simulink model "solar_pv_protected_c07_circuit"  (R2026b)
settings: Solver=VariableStepAuto
model workspace (MAT data in the model file):
  candidate_owner = 'pv_protection_integration_20261023_r01'
  solar_edit_metadata : object (value not decoded)
libraries: fl_lib x149, ee_lib x16, ltc4364demo_lib x3, batteryecm_lib x1, solarprotect_lib x1
(part 13 of 16)

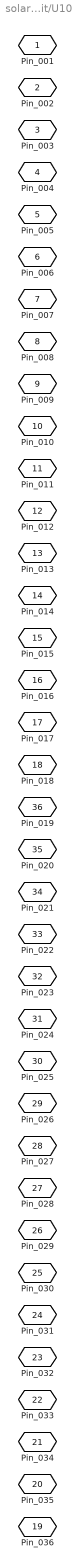
== system solar_pv_protected_c07_circuit/U10 ==
  Pin_001 : PMIOPort  Description=|  Side=Left  ConnectionType=Connection: foundation.electrical.electrical
      | 識別名　　　　　　　; Pin_001
      | 種別　　　　　　　　; Simscape Connection Port（階層境界の物理端子）
      | 所属部品　　　　　　; U10
      | 配置目的　　　　　　; 内部の電気ノードを、この外箱の外側の対応端子へ引き出す。
      | 対応端子　　　　　　; lconn:1／1番 GNDP
      | 接続ラベル　　　　　; GND、PROT_RETURN
      | モデルの範囲　　　　; 実部品を1個追加する表現ではない。端子自体に増幅・遮断・測定機能を持たない。
      | 端子番号の注意　　　; Connection Portの番号は外箱内の対応番号であり、実パッケージのピン番号とは区別する。
      | 確認の範囲　　　　　; 実ポートと階層対応による静的接続の説明。電気特性の再現性は所属部品の説明を参照する。
      | 
      | 従来の補足　　　　　; 以前のDescriptionを以下に保持する。
      | Physical U10 pin 1 / GNDP
      | 
      | 【この説明欄の略語・記号】
      | 用語1　　　　　　　 ; IC：Integrated Circuit（集積回路）。複数の電子素子と機能を小さな半導体チップに集積した部品。
      | 用語2　　　　　　　 ; MOSFET：Metal-Oxide-Semiconductor Field-Effect Transistor（金属・酸化膜・半導体構造の電界効果トランジスタ）。ゲートとソースの電圧でドレインとソースの導通を制御する素子。N-MOSはNチャネル型を表す。
      | 用語3　　　　　　　 ; GND：Ground（回路の基準電位・電流帰路）。この図の共通基準。保護接地や大地への接続を意味するとは限らない。
      | 用語4　　　　　　　 ; VCC/VDD/VEE/VS：ICの電源端子名。文字の歴史的な由来を現在の接続機能へ当てはめない。現回路のVEEはU8/U10では浮動基準SW、U9ではGND。各電圧・基準は端子と接続を参照する。
      | 用語5　　　　　　　 ; GNDP：U10の一次側電源の基準端子。絶縁電源の入力側GND。二次側基準VEE=SWと直接同一の導体ではない。
      | 用語6　　　　　　　 ; SW：Switching Node（スイッチング点）。主電力段の上下MOSFETとL1がつながる、電圧が高速に切り替わる点。GNDとは別電位。
      | 用語7　　　　　　　 ; PROT_RETURN：保護回路の共通帰路。PROTはProtection（保護）、RETURNは帰路。プロトタイプの略ではなく、現回路では共通GNDへつながる。
  Pin_002 : PMIOPort  Description=|  Port=2  Side=Left  ConnectionType=Connection: foundation.electrical.electrical
      | 識別名　　　　　　　; Pin_002
      | 種別　　　　　　　　; Simscape Connection Port（階層境界の物理端子）
      | 所属部品　　　　　　; U10
      | 配置目的　　　　　　; 内部の電気ノードを、この外箱の外側の対応端子へ引き出す。
      | 対応端子　　　　　　; lconn:2／2番 GNDP
      | 接続ラベル　　　　　; GND、PROT_RETURN
      | モデルの範囲　　　　; 実部品を1個追加する表現ではない。端子自体に増幅・遮断・測定機能を持たない。
      | 端子番号の注意　　　; Connection Portの番号は外箱内の対応番号であり、実パッケージのピン番号とは区別する。
      | 確認の範囲　　　　　; 実ポートと階層対応による静的接続の説明。電気特性の再現性は所属部品の説明を参照する。
      | 
      | 従来の補足　　　　　; 以前のDescriptionを以下に保持する。
      | Physical U10 pin 2 / GNDP
      | 
      | 【この説明欄の略語・記号】
      | 用語1　　　　　　　 ; IC：Integrated Circuit（集積回路）。複数の電子素子と機能を小さな半導体チップに集積した部品。
      | 用語2　　　　　　　 ; MOSFET：Metal-Oxide-Semiconductor Field-Effect Transistor（金属・酸化膜・半導体構造の電界効果トランジスタ）。ゲートとソースの電圧でドレインとソースの導通を制御する素子。N-MOSはNチャネル型を表す。
      | 用語3　　　　　　　 ; GND：Ground（回路の基準電位・電流帰路）。この図の共通基準。保護接地や大地への接続を意味するとは限らない。
      | 用語4　　　　　　　 ; VCC/VDD/VEE/VS：ICの電源端子名。文字の歴史的な由来を現在の接続機能へ当てはめない。現回路のVEEはU8/U10では浮動基準SW、U9ではGND。各電圧・基準は端子と接続を参照する。
      | 用語5　　　　　　　 ; GNDP：U10の一次側電源の基準端子。絶縁電源の入力側GND。二次側基準VEE=SWと直接同一の導体ではない。
      | 用語6　　　　　　　 ; SW：Switching Node（スイッチング点）。主電力段の上下MOSFETとL1がつながる、電圧が高速に切り替わる点。GNDとは別電位。
      | 用語7　　　　　　　 ; PROT_RETURN：保護回路の共通帰路。PROTはProtection（保護）、RETURNは帰路。プロトタイプの略ではなく、現回路では共通GNDへつながる。
  Pin_003 : PMIOPort  Description=|  Port=3  Side=Left  ConnectionType=Connection: foundation.electrical.electrical
      | 識別名　　　　　　　; Pin_003
      | 種別　　　　　　　　; Simscape Connection Port（階層境界の物理端子）
      | 所属部品　　　　　　; U10
      | 配置目的　　　　　　; 内部の電気ノードを、この外箱の外側の対応端子へ引き出す。
      | 対応端子　　　　　　; lconn:3／3番 PG
      | 接続ラベル　　　　　; BIAS_PG
      | モデルの範囲　　　　; 実部品を1個追加する表現ではない。端子自体に増幅・遮断・測定機能を持たない。
      | 端子番号の注意　　　; Connection Portの番号は外箱内の対応番号であり、実パッケージのピン番号とは区別する。
      | 確認の範囲　　　　　; 実ポートと階層対応による静的接続の説明。電気特性の再現性は所属部品の説明を参照する。
      | 
      | 従来の補足　　　　　; 以前のDescriptionを以下に保持する。
      | Physical U10 pin 3 / PG
      | 
      | 【この説明欄の略語・記号】
      | 用語1　　　　　　　 ; IC：Integrated Circuit（集積回路）。複数の電子素子と機能を小さな半導体チップに集積した部品。
      | 用語2　　　　　　　 ; PG：Power Good（電源状態通知）。電源出力が規定状態にあるかを知らせる信号。プルアップ条件と実際の通知条件は対象ICの説明で確認する。
  Pin_004 : PMIOPort  Description=|  Port=4  Side=Left  ConnectionType=Connection: foundation.electrical.electrical
      | 識別名　　　　　　　; Pin_004
      | 種別　　　　　　　　; Simscape Connection Port（階層境界の物理端子）
      | 所属部品　　　　　　; U10
      | 配置目的　　　　　　; 内部の電気ノードを、この外箱の外側の対応端子へ引き出す。
      | 対応端子　　　　　　; lconn:4／4番 ENA
      | 接続ラベル　　　　　; BIAS_EN
      | モデルの範囲　　　　; 実部品を1個追加する表現ではない。端子自体に増幅・遮断・測定機能を持たない。
      | 端子番号の注意　　　; Connection Portの番号は外箱内の対応番号であり、実パッケージのピン番号とは区別する。
      | 確認の範囲　　　　　; 実ポートと階層対応による静的接続の説明。電気特性の再現性は所属部品の説明を参照する。
      | 
      | 従来の補足　　　　　; 以前のDescriptionを以下に保持する。
      | Physical U10 pin 4 / ENA
      | 
      | 【この説明欄の略語・記号】
      | 用語1　　　　　　　 ; EN：Enable（動作許可）。対象機能の動作を許可する信号。端子ごとの有効レベルや接続状態に従う。
  Pin_005 : PMIOPort  Description=|  Port=5  Side=Left  ConnectionType=Connection: foundation.electrical.electrical
      | 識別名　　　　　　　; Pin_005
      | 種別　　　　　　　　; Simscape Connection Port（階層境界の物理端子）
      | 所属部品　　　　　　; U10
      | 配置目的　　　　　　; 内部の電気ノードを、この外箱の外側の対応端子へ引き出す。
      | 対応端子　　　　　　; lconn:5／5番 GNDP
      | 接続ラベル　　　　　; GND、PROT_RETURN
      | モデルの範囲　　　　; 実部品を1個追加する表現ではない。端子自体に増幅・遮断・測定機能を持たない。
      | 端子番号の注意　　　; Connection Portの番号は外箱内の対応番号であり、実パッケージのピン番号とは区別する。
      | 確認の範囲　　　　　; 実ポートと階層対応による静的接続の説明。電気特性の再現性は所属部品の説明を参照する。
      | 
      | 従来の補足　　　　　; 以前のDescriptionを以下に保持する。
      | Physical U10 pin 5 / GNDP
      | 
      | 【この説明欄の略語・記号】
      | 用語1　　　　　　　 ; IC：Integrated Circuit（集積回路）。複数の電子素子と機能を小さな半導体チップに集積した部品。
      | 用語2　　　　　　　 ; MOSFET：Metal-Oxide-Semiconductor Field-Effect Transistor（金属・酸化膜・半導体構造の電界効果トランジスタ）。ゲートとソースの電圧でドレインとソースの導通を制御する素子。N-MOSはNチャネル型を表す。
      | 用語3　　　　　　　 ; GND：Ground（回路の基準電位・電流帰路）。この図の共通基準。保護接地や大地への接続を意味するとは限らない。
      | 用語4　　　　　　　 ; VCC/VDD/VEE/VS：ICの電源端子名。文字の歴史的な由来を現在の接続機能へ当てはめない。現回路のVEEはU8/U10では浮動基準SW、U9ではGND。各電圧・基準は端子と接続を参照する。
      | 用語5　　　　　　　 ; GNDP：U10の一次側電源の基準端子。絶縁電源の入力側GND。二次側基準VEE=SWと直接同一の導体ではない。
      | 用語6　　　　　　　 ; SW：Switching Node（スイッチング点）。主電力段の上下MOSFETとL1がつながる、電圧が高速に切り替わる点。GNDとは別電位。
      | 用語7　　　　　　　 ; PROT_RETURN：保護回路の共通帰路。PROTはProtection（保護）、RETURNは帰路。プロトタイプの略ではなく、現回路では共通GNDへつながる。
  Pin_006 : PMIOPort  Description=|  Port=6  Side=Left  ConnectionType=Connection: foundation.electrical.electrical
      | 識別名　　　　　　　; Pin_006
      | 種別　　　　　　　　; Simscape Connection Port（階層境界の物理端子）
      | 所属部品　　　　　　; U10
      | 配置目的　　　　　　; 内部の電気ノードを、この外箱の外側の対応端子へ引き出す。
      | 対応端子　　　　　　; lconn:6／6番 VIN
      | 接続ラベル　　　　　; P12
      | モデルの範囲　　　　; 実部品を1個追加する表現ではない。端子自体に増幅・遮断・測定機能を持たない。
      | 端子番号の注意　　　; Connection Portの番号は外箱内の対応番号であり、実パッケージのピン番号とは区別する。
      | 確認の範囲　　　　　; 実ポートと階層対応による静的接続の説明。電気特性の再現性は所属部品の説明を参照する。
      | 
      | 従来の補足　　　　　; 以前のDescriptionを以下に保持する。
      | Physical U10 pin 6 / VIN
      | 
      | 【この説明欄の略語・記号】
      | 用語1　　　　　　　 ; VIN/VOUT：入力電圧・出力電圧を表す端子／ネット名。INは入力、OUTは出力。電源変換器の電力端子なのか、検出用端子なのかは対象部品によって異なるため、端子と接続の説明に従う。
  Pin_007 : PMIOPort  Description=|  Port=7  Side=Left  ConnectionType=Connection: foundation.electrical.electrical
      | 識別名　　　　　　　; Pin_007
      | 種別　　　　　　　　; Simscape Connection Port（階層境界の物理端子）
      | 所属部品　　　　　　; U10
      | 配置目的　　　　　　; 内部の電気ノードを、この外箱の外側の対応端子へ引き出す。
      | 対応端子　　　　　　; lconn:7／7番 VIN
      | 接続ラベル　　　　　; P12
      | モデルの範囲　　　　; 実部品を1個追加する表現ではない。端子自体に増幅・遮断・測定機能を持たない。
      | 端子番号の注意　　　; Connection Portの番号は外箱内の対応番号であり、実パッケージのピン番号とは区別する。
      | 確認の範囲　　　　　; 実ポートと階層対応による静的接続の説明。電気特性の再現性は所属部品の説明を参照する。
      | 
      | 従来の補足　　　　　; 以前のDescriptionを以下に保持する。
      | Physical U10 pin 7 / VIN
      | 
      | 【この説明欄の略語・記号】
      | 用語1　　　　　　　 ; VIN/VOUT：入力電圧・出力電圧を表す端子／ネット名。INは入力、OUTは出力。電源変換器の電力端子なのか、検出用端子なのかは対象部品によって異なるため、端子と接続の説明に従う。
  Pin_008 : PMIOPort  Description=|  Port=8  Side=Left  ConnectionType=Connection: foundation.electrical.electrical
      | 識別名　　　　　　　; Pin_008
      | 種別　　　　　　　　; Simscape Connection Port（階層境界の物理端子）
      | 所属部品　　　　　　; U10
      | 配置目的　　　　　　; 内部の電気ノードを、この外箱の外側の対応端子へ引き出す。
      | 対応端子　　　　　　; lconn:8／8番 GNDP
      | 接続ラベル　　　　　; GND、PROT_RETURN
      | モデルの範囲　　　　; 実部品を1個追加する表現ではない。端子自体に増幅・遮断・測定機能を持たない。
      | 端子番号の注意　　　; Connection Portの番号は外箱内の対応番号であり、実パッケージのピン番号とは区別する。
      | 確認の範囲　　　　　; 実ポートと階層対応による静的接続の説明。電気特性の再現性は所属部品の説明を参照する。
      | 
      | 従来の補足　　　　　; 以前のDescriptionを以下に保持する。
      | Physical U10 pin 8 / GNDP
      | 
      | 【この説明欄の略語・記号】
      | 用語1　　　　　　　 ; IC：Integrated Circuit（集積回路）。複数の電子素子と機能を小さな半導体チップに集積した部品。
      | 用語2　　　　　　　 ; MOSFET：Metal-Oxide-Semiconductor Field-Effect Transistor（金属・酸化膜・半導体構造の電界効果トランジスタ）。ゲートとソースの電圧でドレインとソースの導通を制御する素子。N-MOSはNチャネル型を表す。
      | 用語3　　　　　　　 ; GND：Ground（回路の基準電位・電流帰路）。この図の共通基準。保護接地や大地への接続を意味するとは限らない。
      | 用語4　　　　　　　 ; VCC/VDD/VEE/VS：ICの電源端子名。文字の歴史的な由来を現在の接続機能へ当てはめない。現回路のVEEはU8/U10では浮動基準SW、U9ではGND。各電圧・基準は端子と接続を参照する。
      | 用語5　　　　　　　 ; GNDP：U10の一次側電源の基準端子。絶縁電源の入力側GND。二次側基準VEE=SWと直接同一の導体ではない。
      | 用語6　　　　　　　 ; SW：Switching Node（スイッチング点）。主電力段の上下MOSFETとL1がつながる、電圧が高速に切り替わる点。GNDとは別電位。
      | 用語7　　　　　　　 ; PROT_RETURN：保護回路の共通帰路。PROTはProtection（保護）、RETURNは帰路。プロトタイプの略ではなく、現回路では共通GNDへつながる。
  Pin_009 : PMIOPort  Description=|  Port=9  Side=Left  ConnectionType=Connection: foundation.electrical.electrical
      | 識別名　　　　　　　; Pin_009
      | 種別　　　　　　　　; Simscape Connection Port（階層境界の物理端子）
      | 所属部品　　　　　　; U10
      | 配置目的　　　　　　; 内部の電気ノードを、この外箱の外側の対応端子へ引き出す。
      | 対応端子　　　　　　; lconn:9／9番 GNDP
      | 接続ラベル　　　　　; GND、PROT_RETURN
      | モデルの範囲　　　　; 実部品を1個追加する表現ではない。端子自体に増幅・遮断・測定機能を持たない。
      | 端子番号の注意　　　; Connection Portの番号は外箱内の対応番号であり、実パッケージのピン番号とは区別する。
      | 確認の範囲　　　　　; 実ポートと階層対応による静的接続の説明。電気特性の再現性は所属部品の説明を参照する。
      | 
      | 従来の補足　　　　　; 以前のDescriptionを以下に保持する。
      | Physical U10 pin 9 / GNDP
      | 
      | 【この説明欄の略語・記号】
      | 用語1　　　　　　　 ; IC：Integrated Circuit（集積回路）。複数の電子素子と機能を小さな半導体チップに集積した部品。
      | 用語2　　　　　　　 ; MOSFET：Metal-Oxide-Semiconductor Field-Effect Transistor（金属・酸化膜・半導体構造の電界効果トランジスタ）。ゲートとソースの電圧でドレインとソースの導通を制御する素子。N-MOSはNチャネル型を表す。
      | 用語3　　　　　　　 ; GND：Ground（回路の基準電位・電流帰路）。この図の共通基準。保護接地や大地への接続を意味するとは限らない。
      | 用語4　　　　　　　 ; VCC/VDD/VEE/VS：ICの電源端子名。文字の歴史的な由来を現在の接続機能へ当てはめない。現回路のVEEはU8/U10では浮動基準SW、U9ではGND。各電圧・基準は端子と接続を参照する。
      | 用語5　　　　　　　 ; GNDP：U10の一次側電源の基準端子。絶縁電源の入力側GND。二次側基準VEE=SWと直接同一の導体ではない。
      | 用語6　　　　　　　 ; SW：Switching Node（スイッチング点）。主電力段の上下MOSFETとL1がつながる、電圧が高速に切り替わる点。GNDとは別電位。
      | 用語7　　　　　　　 ; PROT_RETURN：保護回路の共通帰路。PROTはProtection（保護）、RETURNは帰路。プロトタイプの略ではなく、現回路では共通GNDへつながる。
  Pin_010 : PMIOPort  Description=|  Port=10  Side=Left  ConnectionType=Connection: foundation.electrical.electrical
      | 識別名　　　　　　　; Pin_010
      | 種別　　　　　　　　; Simscape Connection Port（階層境界の物理端子）
      | 所属部品　　　　　　; U10
      | 配置目的　　　　　　; 内部の電気ノードを、この外箱の外側の対応端子へ引き出す。
      | 対応端子　　　　　　; lconn:10／10番 GNDP
      | 接続ラベル　　　　　; GND、PROT_RETURN
      | モデルの範囲　　　　; 実部品を1個追加する表現ではない。端子自体に増幅・遮断・測定機能を持たない。
      | 端子番号の注意　　　; Connection Portの番号は外箱内の対応番号であり、実パッケージのピン番号とは区別する。
      | 確認の範囲　　　　　; 実ポートと階層対応による静的接続の説明。電気特性の再現性は所属部品の説明を参照する。
      | 
      | 従来の補足　　　　　; 以前のDescriptionを以下に保持する。
      | Physical U10 pin 10 / GNDP
      | 
      | 【この説明欄の略語・記号】
      | 用語1　　　　　　　 ; IC：Integrated Circuit（集積回路）。複数の電子素子と機能を小さな半導体チップに集積した部品。
      | 用語2　　　　　　　 ; MOSFET：Metal-Oxide-Semiconductor Field-Effect Transistor（金属・酸化膜・半導体構造の電界効果トランジスタ）。ゲートとソースの電圧でドレインとソースの導通を制御する素子。N-MOSはNチャネル型を表す。
      | 用語3　　　　　　　 ; GND：Ground（回路の基準電位・電流帰路）。この図の共通基準。保護接地や大地への接続を意味するとは限らない。
      | 用語4　　　　　　　 ; VCC/VDD/VEE/VS：ICの電源端子名。文字の歴史的な由来を現在の接続機能へ当てはめない。現回路のVEEはU8/U10では浮動基準SW、U9ではGND。各電圧・基準は端子と接続を参照する。
      | 用語5　　　　　　　 ; GNDP：U10の一次側電源の基準端子。絶縁電源の入力側GND。二次側基準VEE=SWと直接同一の導体ではない。
      | 用語6　　　　　　　 ; SW：Switching Node（スイッチング点）。主電力段の上下MOSFETとL1がつながる、電圧が高速に切り替わる点。GNDとは別電位。
      | 用語7　　　　　　　 ; PROT_RETURN：保護回路の共通帰路。PROTはProtection（保護）、RETURNは帰路。プロトタイプの略ではなく、現回路では共通GNDへつながる。
  Pin_011 : PMIOPort  Description=|  Port=11  Side=Left  ConnectionType=Connection: foundation.electrical.electrical
      | 識別名　　　　　　　; Pin_011
      | 種別　　　　　　　　; Simscape Connection Port（階層境界の物理端子）
      | 所属部品　　　　　　; U10
      | 配置目的　　　　　　; 内部の電気ノードを、この外箱の外側の対応端子へ引き出す。
      | 対応端子　　　　　　; lconn:11／11番 GNDP
      | 接続ラベル　　　　　; GND、PROT_RETURN
      | モデルの範囲　　　　; 実部品を1個追加する表現ではない。端子自体に増幅・遮断・測定機能を持たない。
      | 端子番号の注意　　　; Connection Portの番号は外箱内の対応番号であり、実パッケージのピン番号とは区別する。
      | 確認の範囲　　　　　; 実ポートと階層対応による静的接続の説明。電気特性の再現性は所属部品の説明を参照する。
      | 
      | 従来の補足　　　　　; 以前のDescriptionを以下に保持する。
      | Physical U10 pin 11 / GNDP
      | 
      | 【この説明欄の略語・記号】
      | 用語1　　　　　　　 ; IC：Integrated Circuit（集積回路）。複数の電子素子と機能を小さな半導体チップに集積した部品。
      | 用語2　　　　　　　 ; MOSFET：Metal-Oxide-Semiconductor Field-Effect Transistor（金属・酸化膜・半導体構造の電界効果トランジスタ）。ゲートとソースの電圧でドレインとソースの導通を制御する素子。N-MOSはNチャネル型を表す。
      | 用語3　　　　　　　 ; GND：Ground（回路の基準電位・電流帰路）。この図の共通基準。保護接地や大地への接続を意味するとは限らない。
      | 用語4　　　　　　　 ; VCC/VDD/VEE/VS：ICの電源端子名。文字の歴史的な由来を現在の接続機能へ当てはめない。現回路のVEEはU8/U10では浮動基準SW、U9ではGND。各電圧・基準は端子と接続を参照する。
      | 用語5　　　　　　　 ; GNDP：U10の一次側電源の基準端子。絶縁電源の入力側GND。二次側基準VEE=SWと直接同一の導体ではない。
      | 用語6　　　　　　　 ; SW：Switching Node（スイッチング点）。主電力段の上下MOSFETとL1がつながる、電圧が高速に切り替わる点。GNDとは別電位。
      | 用語7　　　　　　　 ; PROT_RETURN：保護回路の共通帰路。PROTはProtection（保護）、RETURNは帰路。プロトタイプの略ではなく、現回路では共通GNDへつながる。
  Pin_012 : PMIOPort  Description=|  Port=12  Side=Left  ConnectionType=Connection: foundation.electrical.electrical
      | 識別名　　　　　　　; Pin_012
      | 種別　　　　　　　　; Simscape Connection Port（階層境界の物理端子）
      | 所属部品　　　　　　; U10
      | 配置目的　　　　　　; 内部の電気ノードを、この外箱の外側の対応端子へ引き出す。
      | 対応端子　　　　　　; lconn:12／12番 GNDP
      | 接続ラベル　　　　　; GND、PROT_RETURN
      | モデルの範囲　　　　; 実部品を1個追加する表現ではない。端子自体に増幅・遮断・測定機能を持たない。
      | 端子番号の注意　　　; Connection Portの番号は外箱内の対応番号であり、実パッケージのピン番号とは区別する。
      | 確認の範囲　　　　　; 実ポートと階層対応による静的接続の説明。電気特性の再現性は所属部品の説明を参照する。
      | 
      | 従来の補足　　　　　; 以前のDescriptionを以下に保持する。
      | Physical U10 pin 12 / GNDP
      | 
      | 【この説明欄の略語・記号】
      | 用語1　　　　　　　 ; IC：Integrated Circuit（集積回路）。複数の電子素子と機能を小さな半導体チップに集積した部品。
      | 用語2　　　　　　　 ; MOSFET：Metal-Oxide-Semiconductor Field-Effect Transistor（金属・酸化膜・半導体構造の電界効果トランジスタ）。ゲートとソースの電圧でドレインとソースの導通を制御する素子。N-MOSはNチャネル型を表す。
      | 用語3　　　　　　　 ; GND：Ground（回路の基準電位・電流帰路）。この図の共通基準。保護接地や大地への接続を意味するとは限らない。
      | 用語4　　　　　　　 ; VCC/VDD/VEE/VS：ICの電源端子名。文字の歴史的な由来を現在の接続機能へ当てはめない。現回路のVEEはU8/U10では浮動基準SW、U9ではGND。各電圧・基準は端子と接続を参照する。
      | 用語5　　　　　　　 ; GNDP：U10の一次側電源の基準端子。絶縁電源の入力側GND。二次側基準VEE=SWと直接同一の導体ではない。
      | 用語6　　　　　　　 ; SW：Switching Node（スイッチング点）。主電力段の上下MOSFETとL1がつながる、電圧が高速に切り替わる点。GNDとは別電位。
      | 用語7　　　　　　　 ; PROT_RETURN：保護回路の共通帰路。PROTはProtection（保護）、RETURNは帰路。プロトタイプの略ではなく、現回路では共通GNDへつながる。
  Pin_013 : PMIOPort  Description=|  Port=13  Side=Left  ConnectionType=Connection: foundation.electrical.electrical
      | 識別名　　　　　　　; Pin_013
      | 種別　　　　　　　　; Simscape Connection Port（階層境界の物理端子）
      | 所属部品　　　　　　; U10
      | 配置目的　　　　　　; 内部の電気ノードを、この外箱の外側の対応端子へ引き出す。
      | 対応端子　　　　　　; lconn:13／13番 GNDP
      | 接続ラベル　　　　　; GND、PROT_RETURN
      | モデルの範囲　　　　; 実部品を1個追加する表現ではない。端子自体に増幅・遮断・測定機能を持たない。
      | 端子番号の注意　　　; Connection Portの番号は外箱内の対応番号であり、実パッケージのピン番号とは区別する。
      | 確認の範囲　　　　　; 実ポートと階層対応による静的接続の説明。電気特性の再現性は所属部品の説明を参照する。
      | 
      | 従来の補足　　　　　; 以前のDescriptionを以下に保持する。
      | Physical U10 pin 13 / GNDP
      | 
      | 【この説明欄の略語・記号】
      | 用語1　　　　　　　 ; IC：Integrated Circuit（集積回路）。複数の電子素子と機能を小さな半導体チップに集積した部品。
      | 用語2　　　　　　　 ; MOSFET：Metal-Oxide-Semiconductor Field-Effect Transistor（金属・酸化膜・半導体構造の電界効果トランジスタ）。ゲートとソースの電圧でドレインとソースの導通を制御する素子。N-MOSはNチャネル型を表す。
      | 用語3　　　　　　　 ; GND：Ground（回路の基準電位・電流帰路）。この図の共通基準。保護接地や大地への接続を意味するとは限らない。
      | 用語4　　　　　　　 ; VCC/VDD/VEE/VS：ICの電源端子名。文字の歴史的な由来を現在の接続機能へ当てはめない。現回路のVEEはU8/U10では浮動基準SW、U9ではGND。各電圧・基準は端子と接続を参照する。
      | 用語5　　　　　　　 ; GNDP：U10の一次側電源の基準端子。絶縁電源の入力側GND。二次側基準VEE=SWと直接同一の導体ではない。
      | 用語6　　　　　　　 ; SW：Switching Node（スイッチング点）。主電力段の上下MOSFETとL1がつながる、電圧が高速に切り替わる点。GNDとは別電位。
      | 用語7　　　　　　　 ; PROT_RETURN：保護回路の共通帰路。PROTはProtection（保護）、RETURNは帰路。プロトタイプの略ではなく、現回路では共通GNDへつながる。
  Pin_014 : PMIOPort  Description=|  Port=14  Side=Left  ConnectionType=Connection: foundation.electrical.electrical
      | 識別名　　　　　　　; Pin_014
      | 種別　　　　　　　　; Simscape Connection Port（階層境界の物理端子）
      | 所属部品　　　　　　; U10
      | 配置目的　　　　　　; 内部の電気ノードを、この外箱の外側の対応端子へ引き出す。
      | 対応端子　　　　　　; lconn:14／14番 GNDP
      | 接続ラベル　　　　　; GND、PROT_RETURN
      | モデルの範囲　　　　; 実部品を1個追加する表現ではない。端子自体に増幅・遮断・測定機能を持たない。
      | 端子番号の注意　　　; Connection Portの番号は外箱内の対応番号であり、実パッケージのピン番号とは区別する。
      | 確認の範囲　　　　　; 実ポートと階層対応による静的接続の説明。電気特性の再現性は所属部品の説明を参照する。
      | 
      | 従来の補足　　　　　; 以前のDescriptionを以下に保持する。
      | Physical U10 pin 14 / GNDP
      | 
      | 【この説明欄の略語・記号】
      | 用語1　　　　　　　 ; IC：Integrated Circuit（集積回路）。複数の電子素子と機能を小さな半導体チップに集積した部品。
      | 用語2　　　　　　　 ; MOSFET：Metal-Oxide-Semiconductor Field-Effect Transistor（金属・酸化膜・半導体構造の電界効果トランジスタ）。ゲートとソースの電圧でドレインとソースの導通を制御する素子。N-MOSはNチャネル型を表す。
      | 用語3　　　　　　　 ; GND：Ground（回路の基準電位・電流帰路）。この図の共通基準。保護接地や大地への接続を意味するとは限らない。
      | 用語4　　　　　　　 ; VCC/VDD/VEE/VS：ICの電源端子名。文字の歴史的な由来を現在の接続機能へ当てはめない。現回路のVEEはU8/U10では浮動基準SW、U9ではGND。各電圧・基準は端子と接続を参照する。
      | 用語5　　　　　　　 ; GNDP：U10の一次側電源の基準端子。絶縁電源の入力側GND。二次側基準VEE=SWと直接同一の導体ではない。
      | 用語6　　　　　　　 ; SW：Switching Node（スイッチング点）。主電力段の上下MOSFETとL1がつながる、電圧が高速に切り替わる点。GNDとは別電位。
      | 用語7　　　　　　　 ; PROT_RETURN：保護回路の共通帰路。PROTはProtection（保護）、RETURNは帰路。プロトタイプの略ではなく、現回路では共通GNDへつながる。
  Pin_015 : PMIOPort  Description=|  Port=15  Side=Left  ConnectionType=Connection: foundation.electrical.electrical
      | 識別名　　　　　　　; Pin_015
      | 種別　　　　　　　　; Simscape Connection Port（階層境界の物理端子）
      | 所属部品　　　　　　; U10
      | 配置目的　　　　　　; 内部の電気ノードを、この外箱の外側の対応端子へ引き出す。
      | 対応端子　　　　　　; lconn:15／15番 GNDP
      | 接続ラベル　　　　　; GND、PROT_RETURN
      | モデルの範囲　　　　; 実部品を1個追加する表現ではない。端子自体に増幅・遮断・測定機能を持たない。
      | 端子番号の注意　　　; Connection Portの番号は外箱内の対応番号であり、実パッケージのピン番号とは区別する。
      | 確認の範囲　　　　　; 実ポートと階層対応による静的接続の説明。電気特性の再現性は所属部品の説明を参照する。
      | 
      | 従来の補足　　　　　; 以前のDescriptionを以下に保持する。
      | Physical U10 pin 15 / GNDP
      | 
      | 【この説明欄の略語・記号】
      | 用語1　　　　　　　 ; IC：Integrated Circuit（集積回路）。複数の電子素子と機能を小さな半導体チップに集積した部品。
      | 用語2　　　　　　　 ; MOSFET：Metal-Oxide-Semiconductor Field-Effect Transistor（金属・酸化膜・半導体構造の電界効果トランジスタ）。ゲートとソースの電圧でドレインとソースの導通を制御する素子。N-MOSはNチャネル型を表す。
      | 用語3　　　　　　　 ; GND：Ground（回路の基準電位・電流帰路）。この図の共通基準。保護接地や大地への接続を意味するとは限らない。
      | 用語4　　　　　　　 ; VCC/VDD/VEE/VS：ICの電源端子名。文字の歴史的な由来を現在の接続機能へ当てはめない。現回路のVEEはU8/U10では浮動基準SW、U9ではGND。各電圧・基準は端子と接続を参照する。
      | 用語5　　　　　　　 ; GNDP：U10の一次側電源の基準端子。絶縁電源の入力側GND。二次側基準VEE=SWと直接同一の導体ではない。
      | 用語6　　　　　　　 ; SW：Switching Node（スイッチング点）。主電力段の上下MOSFETとL1がつながる、電圧が高速に切り替わる点。GNDとは別電位。
      | 用語7　　　　　　　 ; PROT_RETURN：保護回路の共通帰路。PROTはProtection（保護）、RETURNは帰路。プロトタイプの略ではなく、現回路では共通GNDへつながる。
  Pin_016 : PMIOPort  Description=|  Port=16  Side=Left  ConnectionType=Connection: foundation.electrical.electrical
      | 識別名　　　　　　　; Pin_016
      | 種別　　　　　　　　; Simscape Connection Port（階層境界の物理端子）
      | 所属部品　　　　　　; U10
      | 配置目的　　　　　　; 内部の電気ノードを、この外箱の外側の対応端子へ引き出す。
      | 対応端子　　　　　　; lconn:16／16番 GNDP
      | 接続ラベル　　　　　; GND、PROT_RETURN
      | モデルの範囲　　　　; 実部品を1個追加する表現ではない。端子自体に増幅・遮断・測定機能を持たない。
      | 端子番号の注意　　　; Connection Portの番号は外箱内の対応番号であり、実パッケージのピン番号とは区別する。
      | 確認の範囲　　　　　; 実ポートと階層対応による静的接続の説明。電気特性の再現性は所属部品の説明を参照する。
      | 
      | 従来の補足　　　　　; 以前のDescriptionを以下に保持する。
      | Physical U10 pin 16 / GNDP
      | 
      | 【この説明欄の略語・記号】
      | 用語1　　　　　　　 ; IC：Integrated Circuit（集積回路）。複数の電子素子と機能を小さな半導体チップに集積した部品。
      | 用語2　　　　　　　 ; MOSFET：Metal-Oxide-Semiconductor Field-Effect Transistor（金属・酸化膜・半導体構造の電界効果トランジスタ）。ゲートとソースの電圧でドレインとソースの導通を制御する素子。N-MOSはNチャネル型を表す。
      | 用語3　　　　　　　 ; GND：Ground（回路の基準電位・電流帰路）。この図の共通基準。保護接地や大地への接続を意味するとは限らない。
      | 用語4　　　　　　　 ; VCC/VDD/VEE/VS：ICの電源端子名。文字の歴史的な由来を現在の接続機能へ当てはめない。現回路のVEEはU8/U10では浮動基準SW、U9ではGND。各電圧・基準は端子と接続を参照する。
      | 用語5　　　　　　　 ; GNDP：U10の一次側電源の基準端子。絶縁電源の入力側GND。二次側基準VEE=SWと直接同一の導体ではない。
      | 用語6　　　　　　　 ; SW：Switching Node（スイッチング点）。主電力段の上下MOSFETとL1がつながる、電圧が高速に切り替わる点。GNDとは別電位。
      | 用語7　　　　　　　 ; PROT_RETURN：保護回路の共通帰路。PROTはProtection（保護）、RETURNは帰路。プロトタイプの略ではなく、現回路では共通GNDへつながる。
  Pin_017 : PMIOPort  Description=|  Port=17  Side=Left  ConnectionType=Connection: foundation.electrical.electrical
      | 識別名　　　　　　　; Pin_017
      | 種別　　　　　　　　; Simscape Connection Port（階層境界の物理端子）
      | 所属部品　　　　　　; U10
      | 配置目的　　　　　　; 内部の電気ノードを、この外箱の外側の対応端子へ引き出す。
      | 対応端子　　　　　　; lconn:17／17番 GNDP
      | 接続ラベル　　　　　; GND、PROT_RETURN
      | モデルの範囲　　　　; 実部品を1個追加する表現ではない。端子自体に増幅・遮断・測定機能を持たない。
      | 端子番号の注意　　　; Connection Portの番号は外箱内の対応番号であり、実パッケージのピン番号とは区別する。
      | 確認の範囲　　　　　; 実ポートと階層対応による静的接続の説明。電気特性の再現性は所属部品の説明を参照する。
      | 
      | 従来の補足　　　　　; 以前のDescriptionを以下に保持する。
      | Physical U10 pin 17 / GNDP
      | 
      | 【この説明欄の略語・記号】
      | 用語1　　　　　　　 ; IC：Integrated Circuit（集積回路）。複数の電子素子と機能を小さな半導体チップに集積した部品。
      | 用語2　　　　　　　 ; MOSFET：Metal-Oxide-Semiconductor Field-Effect Transistor（金属・酸化膜・半導体構造の電界効果トランジスタ）。ゲートとソースの電圧でドレインとソースの導通を制御する素子。N-MOSはNチャネル型を表す。
      | 用語3　　　　　　　 ; GND：Ground（回路の基準電位・電流帰路）。この図の共通基準。保護接地や大地への接続を意味するとは限らない。
      | 用語4　　　　　　　 ; VCC/VDD/VEE/VS：ICの電源端子名。文字の歴史的な由来を現在の接続機能へ当てはめない。現回路のVEEはU8/U10では浮動基準SW、U9ではGND。各電圧・基準は端子と接続を参照する。
      | 用語5　　　　　　　 ; GNDP：U10の一次側電源の基準端子。絶縁電源の入力側GND。二次側基準VEE=SWと直接同一の導体ではない。
      | 用語6　　　　　　　 ; SW：Switching Node（スイッチング点）。主電力段の上下MOSFETとL1がつながる、電圧が高速に切り替わる点。GNDとは別電位。
      | 用語7　　　　　　　 ; PROT_RETURN：保護回路の共通帰路。PROTはProtection（保護）、RETURNは帰路。プロトタイプの略ではなく、現回路では共通GNDへつながる。
  Pin_018 : PMIOPort  Description=|  Port=18  Side=Left  ConnectionType=Connection: foundation.electrical.electrical
      | 識別名　　　　　　　; Pin_018
      | 種別　　　　　　　　; Simscape Connection Port（階層境界の物理端子）
      | 所属部品　　　　　　; U10
      | 配置目的　　　　　　; 内部の電気ノードを、この外箱の外側の対応端子へ引き出す。
      | 対応端子　　　　　　; lconn:18／18番 GNDP
      | 接続ラベル　　　　　; GND、PROT_RETURN
      | モデルの範囲　　　　; 実部品を1個追加する表現ではない。端子自体に増幅・遮断・測定機能を持たない。
      | 端子番号の注意　　　; Connection Portの番号は外箱内の対応番号であり、実パッケージのピン番号とは区別する。
      | 確認の範囲　　　　　; 実ポートと階層対応による静的接続の説明。電気特性の再現性は所属部品の説明を参照する。
      | 
      | 従来の補足　　　　　; 以前のDescriptionを以下に保持する。
      | Physical U10 pin 18 / GNDP
      | 
      | 【この説明欄の略語・記号】
      | 用語1　　　　　　　 ; IC：Integrated Circuit（集積回路）。複数の電子素子と機能を小さな半導体チップに集積した部品。
      | 用語2　　　　　　　 ; MOSFET：Metal-Oxide-Semiconductor Field-Effect Transistor（金属・酸化膜・半導体構造の電界効果トランジスタ）。ゲートとソースの電圧でドレインとソースの導通を制御する素子。N-MOSはNチャネル型を表す。
      | 用語3　　　　　　　 ; GND：Ground（回路の基準電位・電流帰路）。この図の共通基準。保護接地や大地への接続を意味するとは限らない。
      | 用語4　　　　　　　 ; VCC/VDD/VEE/VS：ICの電源端子名。文字の歴史的な由来を現在の接続機能へ当てはめない。現回路のVEEはU8/U10では浮動基準SW、U9ではGND。各電圧・基準は端子と接続を参照する。
      | 用語5　　　　　　　 ; GNDP：U10の一次側電源の基準端子。絶縁電源の入力側GND。二次側基準VEE=SWと直接同一の導体ではない。
      | 用語6　　　　　　　 ; SW：Switching Node（スイッチング点）。主電力段の上下MOSFETとL1がつながる、電圧が高速に切り替わる点。GNDとは別電位。
      | 用語7　　　　　　　 ; PROT_RETURN：保護回路の共通帰路。PROTはProtection（保護）、RETURNは帰路。プロトタイプの略ではなく、現回路では共通GNDへつながる。
  Pin_036 : PMIOPort  Description=|  Port=19  Side=Right  ConnectionType=Connection: foundation.electrical.electrical
      | 識別名　　　　　　　; Pin_036
      | 種別　　　　　　　　; Simscape Connection Port（階層境界の物理端子）
      | 所属部品　　　　　　; U10
      | 配置目的　　　　　　; 内部の電気ノードを、この外箱の外側の対応端子へ引き出す。
      | 対応端子　　　　　　; rconn:18／36番 VEE
      | 接続ラベル　　　　　; ラベルなし。接続は実線と境界対応で定義する。
      | モデルの範囲　　　　; 実部品を1個追加する表現ではない。端子自体に増幅・遮断・測定機能を持たない。
      | 端子番号の注意　　　; Connection Portの番号は外箱内の対応番号であり、実パッケージのピン番号とは区別する。
      | 確認の範囲　　　　　; 実ポートと階層対応による静的接続の説明。電気特性の再現性は所属部品の説明を参照する。
      | 
      | 従来の補足　　　　　; 以前のDescriptionを以下に保持する。
      | Physical U10 pin 36 / VEE
      | 
      | 【この説明欄の略語・記号】
      | 用語1　　　　　　　 ; IC：Integrated Circuit（集積回路）。複数の電子素子と機能を小さな半導体チップに集積した部品。
      | 用語2　　　　　　　 ; MOSFET：Metal-Oxide-Semiconductor Field-Effect Transistor（金属・酸化膜・半導体構造の電界効果トランジスタ）。ゲートとソースの電圧でドレインとソースの導通を制御する素子。N-MOSはNチャネル型を表す。
      | 用語3　　　　　　　 ; GND：Ground（回路の基準電位・電流帰路）。この図の共通基準。保護接地や大地への接続を意味するとは限らない。
      | 用語4　　　　　　　 ; VCC/VDD/VEE/VS：ICの電源端子名。文字の歴史的な由来を現在の接続機能へ当てはめない。現回路のVEEはU8/U10では浮動基準SW、U9ではGND。各電圧・基準は端子と接続を参照する。
      | 用語5　　　　　　　 ; SW：Switching Node（スイッチング点）。主電力段の上下MOSFETとL1がつながる、電圧が高速に切り替わる点。GNDとは別電位。
  Pin_035 : PMIOPort  Description=|  Port=20  Side=Right  ConnectionType=Connection: foundation.electrical.electrical
      | 識別名　　　　　　　; Pin_035
      | 種別　　　　　　　　; Simscape Connection Port（階層境界の物理端子）
      | 所属部品　　　　　　; U10
      | 配置目的　　　　　　; 内部の電気ノードを、この外箱の外側の対応端子へ引き出す。
      | 対応端子　　　　　　; rconn:17／35番 VEEA
      | 接続ラベル　　　　　; ラベルなし。接続は実線と境界対応で定義する。
      | モデルの範囲　　　　; 実部品を1個追加する表現ではない。端子自体に増幅・遮断・測定機能を持たない。
      | 端子番号の注意　　　; Connection Portの番号は外箱内の対応番号であり、実パッケージのピン番号とは区別する。
      | 確認の範囲　　　　　; 実ポートと階層対応による静的接続の説明。電気特性の再現性は所属部品の説明を参照する。
      | 
      | 従来の補足　　　　　; 以前のDescriptionを以下に保持する。
      | Physical U10 pin 35 / VEEA
      | 
      | 【この説明欄の略語・記号】
      | 用語1　　　　　　　 ; MOSFET：Metal-Oxide-Semiconductor Field-Effect Transistor（金属・酸化膜・半導体構造の電界効果トランジスタ）。ゲートとソースの電圧でドレインとソースの導通を制御する素子。N-MOSはNチャネル型を表す。
      | 用語2　　　　　　　 ; GND：Ground（回路の基準電位・電流帰路）。この図の共通基準。保護接地や大地への接続を意味するとは限らない。
      | 用語3　　　　　　　 ; VEEA：U10の二次側アナログ基準端子。現回路ではSWへ接続する。共通GNDへ接続する意味ではない。
      | 用語4　　　　　　　 ; SW：Switching Node（スイッチング点）。主電力段の上下MOSFETとL1がつながる、電圧が高速に切り替わる点。GNDとは別電位。
  Pin_034 : PMIOPort  Description=|  Port=21  Side=Right  ConnectionType=Connection: foundation.electrical.electrical
      | 識別名　　　　　　　; Pin_034
      | 種別　　　　　　　　; Simscape Connection Port（階層境界の物理端子）
      | 所属部品　　　　　　; U10
      | 配置目的　　　　　　; 内部の電気ノードを、この外箱の外側の対応端子へ引き出す。
      | 対応端子　　　　　　; rconn:16／34番 FBVDD
      | 接続ラベル　　　　　; H_FB
      | モデルの範囲　　　　; 実部品を1個追加する表現ではない。端子自体に増幅・遮断・測定機能を持たない。
      | 端子番号の注意　　　; Connection Portの番号は外箱内の対応番号であり、実パッケージのピン番号とは区別する。
      | 確認の範囲　　　　　; 実ポートと階層対応による静的接続の説明。電気特性の再現性は所属部品の説明を参照する。
      | 
      | 従来の補足　　　　　; 以前のDescriptionを以下に保持する。
      | Physical U10 pin 34 / FBVDD
      | 
      | 【この説明欄の略語・記号】
      | 用語1　　　　　　　 ; FB：Feedback（帰還）。出力などを検出して内部制御へ戻すための信号・端子。
      | 用語2　　　　　　　 ; FBVDD/FBVEE：U10の出力電圧帰還端子。二次側の出力電圧設定に用いる。現接続では両端子がH_FBへ接続される。
  Pin_033 : PMIOPort  Description=|  Port=22  Side=Right  ConnectionType=Connection: foundation.electrical.electrical
      | 識別名　　　　　　　; Pin_033
      | 種別　　　　　　　　; Simscape Connection Port（階層境界の物理端子）
      | 所属部品　　　　　　; U10
      | 配置目的　　　　　　; 内部の電気ノードを、この外箱の外側の対応端子へ引き出す。
      | 対応端子　　　　　　; rconn:15／33番 FBVEE
      | 接続ラベル　　　　　; H_FB
      | モデルの範囲　　　　; 実部品を1個追加する表現ではない。端子自体に増幅・遮断・測定機能を持たない。
      | 端子番号の注意　　　; Connection Portの番号は外箱内の対応番号であり、実パッケージのピン番号とは区別する。
      | 確認の範囲　　　　　; 実ポートと階層対応による静的接続の説明。電気特性の再現性は所属部品の説明を参照する。
      | 
      | 従来の補足　　　　　; 以前のDescriptionを以下に保持する。
      | Physical U10 pin 33 / FBVEE
      | 
      | 【この説明欄の略語・記号】
      | 用語1　　　　　　　 ; FB：Feedback（帰還）。出力などを検出して内部制御へ戻すための信号・端子。
      | 用語2　　　　　　　 ; FBVDD/FBVEE：U10の出力電圧帰還端子。二次側の出力電圧設定に用いる。現接続では両端子がH_FBへ接続される。
  Pin_032 : PMIOPort  Description=|  Port=23  Side=Right  ConnectionType=Connection: foundation.electrical.electrical
      | 識別名　　　　　　　; Pin_032
      | 種別　　　　　　　　; Simscape Connection Port（階層境界の物理端子）
      | 所属部品　　　　　　; U10
      | 配置目的　　　　　　; 内部の電気ノードを、この外箱の外側の対応端子へ引き出す。
      | 対応端子　　　　　　; rconn:14／32番 RLIM
      | 接続ラベル　　　　　; ラベルなし。接続は実線と境界対応で定義する。
      | モデルの範囲　　　　; 実部品を1個追加する表現ではない。端子自体に増幅・遮断・測定機能を持たない。
      | 端子番号の注意　　　; Connection Portの番号は外箱内の対応番号であり、実パッケージのピン番号とは区別する。
      | 確認の範囲　　　　　; 実ポートと階層対応による静的接続の説明。電気特性の再現性は所属部品の説明を参照する。
      | 
      | 従来の補足　　　　　; 以前のDescriptionを以下に保持する。
      | Physical U10 pin 32 / RLIM
      | 
      | 【この説明欄の略語・記号】
      | 用語1　　　　　　　 ; RLIM：U10の外付け抵抗による制限設定端子。外付けR47で二次側の電圧調整に使う電流を制限する端子。主電力段の充電電流制限とは別の機能。
  Pin_031 : PMIOPort  Description=|  Port=24  Side=Right  ConnectionType=Connection: foundation.electrical.electrical
      | 識別名　　　　　　　; Pin_031
      | 種別　　　　　　　　; Simscape Connection Port（階層境界の物理端子）
      | 所属部品　　　　　　; U10
      | 配置目的　　　　　　; 内部の電気ノードを、この外箱の外側の対応端子へ引き出す。
      | 対応端子　　　　　　; rconn:13／31番 VEE
      | 接続ラベル　　　　　; ラベルなし。接続は実線と境界対応で定義する。
      | モデルの範囲　　　　; 実部品を1個追加する表現ではない。端子自体に増幅・遮断・測定機能を持たない。
      | 端子番号の注意　　　; Connection Portの番号は外箱内の対応番号であり、実パッケージのピン番号とは区別する。
      | 確認の範囲　　　　　; 実ポートと階層対応による静的接続の説明。電気特性の再現性は所属部品の説明を参照する。
      | 
      | 従来の補足　　　　　; 以前のDescriptionを以下に保持する。
      | Physical U10 pin 31 / VEE
      | 
      | 【この説明欄の略語・記号】
      | 用語1　　　　　　　 ; IC：Integrated Circuit（集積回路）。複数の電子素子と機能を小さな半導体チップに集積した部品。
      | 用語2　　　　　　　 ; MOSFET：Metal-Oxide-Semiconductor Field-Effect Transistor（金属・酸化膜・半導体構造の電界効果トランジスタ）。ゲートとソースの電圧でドレインとソースの導通を制御する素子。N-MOSはNチャネル型を表す。
      | 用語3　　　　　　　 ; GND：Ground（回路の基準電位・電流帰路）。この図の共通基準。保護接地や大地への接続を意味するとは限らない。
      | 用語4　　　　　　　 ; VCC/VDD/VEE/VS：ICの電源端子名。文字の歴史的な由来を現在の接続機能へ当てはめない。現回路のVEEはU8/U10では浮動基準SW、U9ではGND。各電圧・基準は端子と接続を参照する。
      | 用語5　　　　　　　 ; SW：Switching Node（スイッチング点）。主電力段の上下MOSFETとL1がつながる、電圧が高速に切り替わる点。GNDとは別電位。
  Pin_030 : PMIOPort  Description=|  Port=25  Side=Right  ConnectionType=Connection: foundation.electrical.electrical
      | 識別名　　　　　　　; Pin_030
      | 種別　　　　　　　　; Simscape Connection Port（階層境界の物理端子）
      | 所属部品　　　　　　; U10
      | 配置目的　　　　　　; 内部の電気ノードを、この外箱の外側の対応端子へ引き出す。
      | 対応端子　　　　　　; rconn:12／30番 VEE
      | 接続ラベル　　　　　; ラベルなし。接続は実線と境界対応で定義する。
      | モデルの範囲　　　　; 実部品を1個追加する表現ではない。端子自体に増幅・遮断・測定機能を持たない。
      | 端子番号の注意　　　; Connection Portの番号は外箱内の対応番号であり、実パッケージのピン番号とは区別する。
      | 確認の範囲　　　　　; 実ポートと階層対応による静的接続の説明。電気特性の再現性は所属部品の説明を参照する。
      | 
      | 従来の補足　　　　　; 以前のDescriptionを以下に保持する。
      | Physical U10 pin 30 / VEE
      | 
      | 【この説明欄の略語・記号】
      | 用語1　　　　　　　 ; IC：Integrated Circuit（集積回路）。複数の電子素子と機能を小さな半導体チップに集積した部品。
      | 用語2　　　　　　　 ; MOSFET：Metal-Oxide-Semiconductor Field-Effect Transistor（金属・酸化膜・半導体構造の電界効果トランジスタ）。ゲートとソースの電圧でドレインとソースの導通を制御する素子。N-MOSはNチャネル型を表す。
      | 用語3　　　　　　　 ; GND：Ground（回路の基準電位・電流帰路）。この図の共通基準。保護接地や大地への接続を意味するとは限らない。
      | 用語4　　　　　　　 ; VCC/VDD/VEE/VS：ICの電源端子名。文字の歴史的な由来を現在の接続機能へ当てはめない。現回路のVEEはU8/U10では浮動基準SW、U9ではGND。各電圧・基準は端子と接続を参照する。
      | 用語5　　　　　　　 ; SW：Switching Node（スイッチング点）。主電力段の上下MOSFETとL1がつながる、電圧が高速に切り替わる点。GNDとは別電位。
  Pin_029 : PMIOPort  Description=|  Port=26  Side=Right  ConnectionType=Connection: foundation.electrical.electrical
      | 識別名　　　　　　　; Pin_029
      | 種別　　　　　　　　; Simscape Connection Port（階層境界の物理端子）
      | 所属部品　　　　　　; U10
      | 配置目的　　　　　　; 内部の電気ノードを、この外箱の外側の対応端子へ引き出す。
      | 対応端子　　　　　　; rconn:11／29番 VDD
      | 接続ラベル　　　　　; H12
      | モデルの範囲　　　　; 実部品を1個追加する表現ではない。端子自体に増幅・遮断・測定機能を持たない。
      | 端子番号の注意　　　; Connection Portの番号は外箱内の対応番号であり、実パッケージのピン番号とは区別する。
      | 確認の範囲　　　　　; 実ポートと階層対応による静的接続の説明。電気特性の再現性は所属部品の説明を参照する。
      | 
      | 従来の補足　　　　　; 以前のDescriptionを以下に保持する。
      | Physical U10 pin 29 / VDD
      | 
      | 【この説明欄の略語・記号】
      | 用語1　　　　　　　 ; IC：Integrated Circuit（集積回路）。複数の電子素子と機能を小さな半導体チップに集積した部品。
      | 用語2　　　　　　　 ; MOSFET：Metal-Oxide-Semiconductor Field-Effect Transistor（金属・酸化膜・半導体構造の電界効果トランジスタ）。ゲートとソースの電圧でドレインとソースの導通を制御する素子。N-MOSはNチャネル型を表す。
      | 用語3　　　　　　　 ; GND：Ground（回路の基準電位・電流帰路）。この図の共通基準。保護接地や大地への接続を意味するとは限らない。
      | 用語4　　　　　　　 ; VCC/VDD/VEE/VS：ICの電源端子名。文字の歴史的な由来を現在の接続機能へ当てはめない。現回路のVEEはU8/U10では浮動基準SW、U9ではGND。各電圧・基準は端子と接続を参照する。
      | 用語5　　　　　　　 ; SW：Switching Node（スイッチング点）。主電力段の上下MOSFETとL1がつながる、電圧が高速に切り替わる点。GNDとは別電位。
  Pin_028 : PMIOPort  Description=|  Port=27  Side=Right  ConnectionType=Connection: foundation.electrical.electrical
      | 識別名　　　　　　　; Pin_028
      | 種別　　　　　　　　; Simscape Connection Port（階層境界の物理端子）
      | 所属部品　　　　　　; U10
      | 配置目的　　　　　　; 内部の電気ノードを、この外箱の外側の対応端子へ引き出す。
      | 対応端子　　　　　　; rconn:10／28番 VDD
      | 接続ラベル　　　　　; H12
      | モデルの範囲　　　　; 実部品を1個追加する表現ではない。端子自体に増幅・遮断・測定機能を持たない。
      | 端子番号の注意　　　; Connection Portの番号は外箱内の対応番号であり、実パッケージのピン番号とは区別する。
      | 確認の範囲　　　　　; 実ポートと階層対応による静的接続の説明。電気特性の再現性は所属部品の説明を参照する。
      | 
      | 従来の補足　　　　　; 以前のDescriptionを以下に保持する。
      | Physical U10 pin 28 / VDD
      | 
      | 【この説明欄の略語・記号】
      | 用語1　　　　　　　 ; IC：Integrated Circuit（集積回路）。複数の電子素子と機能を小さな半導体チップに集積した部品。
      | 用語2　　　　　　　 ; MOSFET：Metal-Oxide-Semiconductor Field-Effect Transistor（金属・酸化膜・半導体構造の電界効果トランジスタ）。ゲートとソースの電圧でドレインとソースの導通を制御する素子。N-MOSはNチャネル型を表す。
      | 用語3　　　　　　　 ; GND：Ground（回路の基準電位・電流帰路）。この図の共通基準。保護接地や大地への接続を意味するとは限らない。
      | 用語4　　　　　　　 ; VCC/VDD/VEE/VS：ICの電源端子名。文字の歴史的な由来を現在の接続機能へ当てはめない。現回路のVEEはU8/U10では浮動基準SW、U9ではGND。各電圧・基準は端子と接続を参照する。
      | 用語5　　　　　　　 ; SW：Switching Node（スイッチング点）。主電力段の上下MOSFETとL1がつながる、電圧が高速に切り替わる点。GNDとは別電位。
  Pin_027 : PMIOPort  Description=|  Port=28  Side=Right  ConnectionType=Connection: foundation.electrical.electrical
      | 識別名　　　　　　　; Pin_027
      | 種別　　　　　　　　; Simscape Connection Port（階層境界の物理端子）
      | 所属部品　　　　　　; U10
      | 配置目的　　　　　　; 内部の電気ノードを、この外箱の外側の対応端子へ引き出す。
      | 対応端子　　　　　　; rconn:9／27番 VEE
      | 接続ラベル　　　　　; ラベルなし。接続は実線と境界対応で定義する。
      | モデルの範囲　　　　; 実部品を1個追加する表現ではない。端子自体に増幅・遮断・測定機能を持たない。
      | 端子番号の注意　　　; Connection Portの番号は外箱内の対応番号であり、実パッケージのピン番号とは区別する。
      | 確認の範囲　　　　　; 実ポートと階層対応による静的接続の説明。電気特性の再現性は所属部品の説明を参照する。
      | 
      | 従来の補足　　　　　; 以前のDescriptionを以下に保持する。
      | Physical U10 pin 27 / VEE
      | 
      | 【この説明欄の略語・記号】
      | 用語1　　　　　　　 ; IC：Integrated Circuit（集積回路）。複数の電子素子と機能を小さな半導体チップに集積した部品。
      | 用語2　　　　　　　 ; MOSFET：Metal-Oxide-Semiconductor Field-Effect Transistor（金属・酸化膜・半導体構造の電界効果トランジスタ）。ゲートとソースの電圧でドレインとソースの導通を制御する素子。N-MOSはNチャネル型を表す。
      | 用語3　　　　　　　 ; GND：Ground（回路の基準電位・電流帰路）。この図の共通基準。保護接地や大地への接続を意味するとは限らない。
      | 用語4　　　　　　　 ; VCC/VDD/VEE/VS：ICの電源端子名。文字の歴史的な由来を現在の接続機能へ当てはめない。現回路のVEEはU8/U10では浮動基準SW、U9ではGND。各電圧・基準は端子と接続を参照する。
      | 用語5　　　　　　　 ; SW：Switching Node（スイッチング点）。主電力段の上下MOSFETとL1がつながる、電圧が高速に切り替わる点。GNDとは別電位。
  Pin_026 : PMIOPort  Description=|  Port=29  Side=Right  ConnectionType=Connection: foundation.electrical.electrical
      | 識別名　　　　　　　; Pin_026
      | 種別　　　　　　　　; Simscape Connection Port（階層境界の物理端子）
      | 所属部品　　　　　　; U10
      | 配置目的　　　　　　; 内部の電気ノードを、この外箱の外側の対応端子へ引き出す。
      | 対応端子　　　　　　; rconn:8／26番 VEE
      | 接続ラベル　　　　　; ラベルなし。接続は実線と境界対応で定義する。
      | モデルの範囲　　　　; 実部品を1個追加する表現ではない。端子自体に増幅・遮断・測定機能を持たない。
      | 端子番号の注意　　　; Connection Portの番号は外箱内の対応番号であり、実パッケージのピン番号とは区別する。
      | 確認の範囲　　　　　; 実ポートと階層対応による静的接続の説明。電気特性の再現性は所属部品の説明を参照する。
      | 
      | 従来の補足　　　　　; 以前のDescriptionを以下に保持する。
      | Physical U10 pin 26 / VEE
      | 
      | 【この説明欄の略語・記号】
      | 用語1　　　　　　　 ; IC：Integrated Circuit（集積回路）。複数の電子素子と機能を小さな半導体チップに集積した部品。
      | 用語2　　　　　　　 ; MOSFET：Metal-Oxide-Semiconductor Field-Effect Transistor（金属・酸化膜・半導体構造の電界効果トランジスタ）。ゲートとソースの電圧でドレインとソースの導通を制御する素子。N-MOSはNチャネル型を表す。
      | 用語3　　　　　　　 ; GND：Ground（回路の基準電位・電流帰路）。この図の共通基準。保護接地や大地への接続を意味するとは限らない。
      | 用語4　　　　　　　 ; VCC/VDD/VEE/VS：ICの電源端子名。文字の歴史的な由来を現在の接続機能へ当てはめない。現回路のVEEはU8/U10では浮動基準SW、U9ではGND。各電圧・基準は端子と接続を参照する。
      | 用語5　　　　　　　 ; SW：Switching Node（スイッチング点）。主電力段の上下MOSFETとL1がつながる、電圧が高速に切り替わる点。GNDとは別電位。
  Pin_025 : PMIOPort  Description=|  Port=30  Side=Right  ConnectionType=Connection: foundation.electrical.electrical
      | 識別名　　　　　　　; Pin_025
      | 種別　　　　　　　　; Simscape Connection Port（階層境界の物理端子）
      | 所属部品　　　　　　; U10
      | 配置目的　　　　　　; 内部の電気ノードを、この外箱の外側の対応端子へ引き出す。
      | 対応端子　　　　　　; rconn:7／25番 VEE
      | 接続ラベル　　　　　; ラベルなし。接続は実線と境界対応で定義する。
      | モデルの範囲　　　　; 実部品を1個追加する表現ではない。端子自体に増幅・遮断・測定機能を持たない。
      | 端子番号の注意　　　; Connection Portの番号は外箱内の対応番号であり、実パッケージのピン番号とは区別する。
      | 確認の範囲　　　　　; 実ポートと階層対応による静的接続の説明。電気特性の再現性は所属部品の説明を参照する。
      | 
      | 従来の補足　　　　　; 以前のDescriptionを以下に保持する。
      | Physical U10 pin 25 / VEE
      | 
      | 【この説明欄の略語・記号】
      | 用語1　　　　　　　 ; IC：Integrated Circuit（集積回路）。複数の電子素子と機能を小さな半導体チップに集積した部品。
      | 用語2　　　　　　　 ; MOSFET：Metal-Oxide-Semiconductor Field-Effect Transistor（金属・酸化膜・半導体構造の電界効果トランジスタ）。ゲートとソースの電圧でドレインとソースの導通を制御する素子。N-MOSはNチャネル型を表す。
      | 用語3　　　　　　　 ; GND：Ground（回路の基準電位・電流帰路）。この図の共通基準。保護接地や大地への接続を意味するとは限らない。
      | 用語4　　　　　　　 ; VCC/VDD/VEE/VS：ICの電源端子名。文字の歴史的な由来を現在の接続機能へ当てはめない。現回路のVEEはU8/U10では浮動基準SW、U9ではGND。各電圧・基準は端子と接続を参照する。
      | 用語5　　　　　　　 ; SW：Switching Node（スイッチング点）。主電力段の上下MOSFETとL1がつながる、電圧が高速に切り替わる点。GNDとは別電位。
  Pin_024 : PMIOPort  Description=|  Port=31  Side=Right  ConnectionType=Connection: foundation.electrical.electrical
      | 識別名　　　　　　　; Pin_024
      | 種別　　　　　　　　; Simscape Connection Port（階層境界の物理端子）
      | 所属部品　　　　　　; U10
      | 配置目的　　　　　　; 内部の電気ノードを、この外箱の外側の対応端子へ引き出す。
      | 対応端子　　　　　　; rconn:6／24番 VEE
      | 接続ラベル　　　　　; ラベルなし。接続は実線と境界対応で定義する。
      | モデルの範囲　　　　; 実部品を1個追加する表現ではない。端子自体に増幅・遮断・測定機能を持たない。
      | 端子番号の注意　　　; Connection Portの番号は外箱内の対応番号であり、実パッケージのピン番号とは区別する。
      | 確認の範囲　　　　　; 実ポートと階層対応による静的接続の説明。電気特性の再現性は所属部品の説明を参照する。
      | 
      | 従来の補足　　　　　; 以前のDescriptionを以下に保持する。
      | Physical U10 pin 24 / VEE
      | 
      | 【この説明欄の略語・記号】
      | 用語1　　　　　　　 ; IC：Integrated Circuit（集積回路）。複数の電子素子と機能を小さな半導体チップに集積した部品。
      | 用語2　　　　　　　 ; MOSFET：Metal-Oxide-Semiconductor Field-Effect Transistor（金属・酸化膜・半導体構造の電界効果トランジスタ）。ゲートとソースの電圧でドレインとソースの導通を制御する素子。N-MOSはNチャネル型を表す。
      | 用語3　　　　　　　 ; GND：Ground（回路の基準電位・電流帰路）。この図の共通基準。保護接地や大地への接続を意味するとは限らない。
      | 用語4　　　　　　　 ; VCC/VDD/VEE/VS：ICの電源端子名。文字の歴史的な由来を現在の接続機能へ当てはめない。現回路のVEEはU8/U10では浮動基準SW、U9ではGND。各電圧・基準は端子と接続を参照する。
      | 用語5　　　　　　　 ; SW：Switching Node（スイッチング点）。主電力段の上下MOSFETとL1がつながる、電圧が高速に切り替わる点。GNDとは別電位。
  Pin_023 : PMIOPort  Description=|  Port=32  Side=Right  ConnectionType=Connection: foundation.electrical.electrical
      | 識別名　　　　　　　; Pin_023
      | 種別　　　　　　　　; Simscape Connection Port（階層境界の物理端子）
      | 所属部品　　　　　　; U10
      | 配置目的　　　　　　; 内部の電気ノードを、この外箱の外側の対応端子へ引き出す。
      | 対応端子　　　　　　; rconn:5／23番 VEE
      | 接続ラベル　　　　　; ラベルなし。接続は実線と境界対応で定義する。
      | モデルの範囲　　　　; 実部品を1個追加する表現ではない。端子自体に増幅・遮断・測定機能を持たない。
      | 端子番号の注意　　　; Connection Portの番号は外箱内の対応番号であり、実パッケージのピン番号とは区別する。
      | 確認の範囲　　　　　; 実ポートと階層対応による静的接続の説明。電気特性の再現性は所属部品の説明を参照する。
      | 
      | 従来の補足　　　　　; 以前のDescriptionを以下に保持する。
      | Physical U10 pin 23 / VEE
      | 
      | 【この説明欄の略語・記号】
      | 用語1　　　　　　　 ; IC：Integrated Circuit（集積回路）。複数の電子素子と機能を小さな半導体チップに集積した部品。
      | 用語2　　　　　　　 ; MOSFET：Metal-Oxide-Semiconductor Field-Effect Transistor（金属・酸化膜・半導体構造の電界効果トランジスタ）。ゲートとソースの電圧でドレインとソースの導通を制御する素子。N-MOSはNチャネル型を表す。
      | 用語3　　　　　　　 ; GND：Ground（回路の基準電位・電流帰路）。この図の共通基準。保護接地や大地への接続を意味するとは限らない。
      | 用語4　　　　　　　 ; VCC/VDD/VEE/VS：ICの電源端子名。文字の歴史的な由来を現在の接続機能へ当てはめない。現回路のVEEはU8/U10では浮動基準SW、U9ではGND。各電圧・基準は端子と接続を参照する。
      | 用語5　　　　　　　 ; SW：Switching Node（スイッチング点）。主電力段の上下MOSFETとL1がつながる、電圧が高速に切り替わる点。GNDとは別電位。
  Pin_022 : PMIOPort  Description=|  Port=33  Side=Right  ConnectionType=Connection: foundation.electrical.electrical
      | 識別名　　　　　　　; Pin_022
      | 種別　　　　　　　　; Simscape Connection Port（階層境界の物理端子）
      | 所属部品　　　　　　; U10
      | 配置目的　　　　　　; 内部の電気ノードを、この外箱の外側の対応端子へ引き出す。
      | 対応端子　　　　　　; rconn:4／22番 VEE
      | 接続ラベル　　　　　; ラベルなし。接続は実線と境界対応で定義する。
      | モデルの範囲　　　　; 実部品を1個追加する表現ではない。端子自体に増幅・遮断・測定機能を持たない。
      | 端子番号の注意　　　; Connection Portの番号は外箱内の対応番号であり、実パッケージのピン番号とは区別する。
      | 確認の範囲　　　　　; 実ポートと階層対応による静的接続の説明。電気特性の再現性は所属部品の説明を参照する。
      | 
      | 従来の補足　　　　　; 以前のDescriptionを以下に保持する。
      | Physical U10 pin 22 / VEE
      | 
      | 【この説明欄の略語・記号】
      | 用語1　　　　　　　 ; IC：Integrated Circuit（集積回路）。複数の電子素子と機能を小さな半導体チップに集積した部品。
      | 用語2　　　　　　　 ; MOSFET：Metal-Oxide-Semiconductor Field-Effect Transistor（金属・酸化膜・半導体構造の電界効果トランジスタ）。ゲートとソースの電圧でドレインとソースの導通を制御する素子。N-MOSはNチャネル型を表す。
      | 用語3　　　　　　　 ; GND：Ground（回路の基準電位・電流帰路）。この図の共通基準。保護接地や大地への接続を意味するとは限らない。
      | 用語4　　　　　　　 ; VCC/VDD/VEE/VS：ICの電源端子名。文字の歴史的な由来を現在の接続機能へ当てはめない。現回路のVEEはU8/U10では浮動基準SW、U9ではGND。各電圧・基準は端子と接続を参照する。
      | 用語5　　　　　　　 ; SW：Switching Node（スイッチング点）。主電力段の上下MOSFETとL1がつながる、電圧が高速に切り替わる点。GNDとは別電位。
  Pin_021 : PMIOPort  Description=|  Port=34  Side=Right  ConnectionType=Connection: foundation.electrical.electrical
      | 識別名　　　　　　　; Pin_021
      | 種別　　　　　　　　; Simscape Connection Port（階層境界の物理端子）
      | 所属部品　　　　　　; U10
      | 配置目的　　　　　　; 内部の電気ノードを、この外箱の外側の対応端子へ引き出す。
      | 対応端子　　　　　　; rconn:3／21番 VEE
      | 接続ラベル　　　　　; ラベルなし。接続は実線と境界対応で定義する。
      | モデルの範囲　　　　; 実部品を1個追加する表現ではない。端子自体に増幅・遮断・測定機能を持たない。
      | 端子番号の注意　　　; Connection Portの番号は外箱内の対応番号であり、実パッケージのピン番号とは区別する。
      | 確認の範囲　　　　　; 実ポートと階層対応による静的接続の説明。電気特性の再現性は所属部品の説明を参照する。
      | 
      | 従来の補足　　　　　; 以前のDescriptionを以下に保持する。
      | Physical U10 pin 21 / VEE
      | 
      | 【この説明欄の略語・記号】
      | 用語1　　　　　　　 ; IC：Integrated Circuit（集積回路）。複数の電子素子と機能を小さな半導体チップに集積した部品。
      | 用語2　　　　　　　 ; MOSFET：Metal-Oxide-Semiconductor Field-Effect Transistor（金属・酸化膜・半導体構造の電界効果トランジスタ）。ゲートとソースの電圧でドレインとソースの導通を制御する素子。N-MOSはNチャネル型を表す。
      | 用語3　　　　　　　 ; GND：Ground（回路の基準電位・電流帰路）。この図の共通基準。保護接地や大地への接続を意味するとは限らない。
      | 用語4　　　　　　　 ; VCC/VDD/VEE/VS：ICの電源端子名。文字の歴史的な由来を現在の接続機能へ当てはめない。現回路のVEEはU8/U10では浮動基準SW、U9ではGND。各電圧・基準は端子と接続を参照する。
      | 用語5　　　　　　　 ; SW：Switching Node（スイッチング点）。主電力段の上下MOSFETとL1がつながる、電圧が高速に切り替わる点。GNDとは別電位。
  Pin_020 : PMIOPort  Description=|  Port=35  Side=Right  ConnectionType=Connection: foundation.electrical.electrical
      | 識別名　　　　　　　; Pin_020
      | 種別　　　　　　　　; Simscape Connection Port（階層境界の物理端子）
      | 所属部品　　　　　　; U10
      | 配置目的　　　　　　; 内部の電気ノードを、この外箱の外側の対応端子へ引き出す。
      | 対応端子　　　　　　; rconn:2／20番 VEE
      | 接続ラベル　　　　　; ラベルなし。接続は実線と境界対応で定義する。
      | モデルの範囲　　　　; 実部品を1個追加する表現ではない。端子自体に増幅・遮断・測定機能を持たない。
      | 端子番号の注意　　　; Connection Portの番号は外箱内の対応番号であり、実パッケージのピン番号とは区別する。
      | 確認の範囲　　　　　; 実ポートと階層対応による静的接続の説明。電気特性の再現性は所属部品の説明を参照する。
      | 
      | 従来の補足　　　　　; 以前のDescriptionを以下に保持する。
      | Physical U10 pin 20 / VEE
      | 
      | 【この説明欄の略語・記号】
      | 用語1　　　　　　　 ; IC：Integrated Circuit（集積回路）。複数の電子素子と機能を小さな半導体チップに集積した部品。
      | 用語2　　　　　　　 ; MOSFET：Metal-Oxide-Semiconductor Field-Effect Transistor（金属・酸化膜・半導体構造の電界効果トランジスタ）。ゲートとソースの電圧でドレインとソースの導通を制御する素子。N-MOSはNチャネル型を表す。
      | 用語3　　　　　　　 ; GND：Ground（回路の基準電位・電流帰路）。この図の共通基準。保護接地や大地への接続を意味するとは限らない。
      | 用語4　　　　　　　 ; VCC/VDD/VEE/VS：ICの電源端子名。文字の歴史的な由来を現在の接続機能へ当てはめない。現回路のVEEはU8/U10では浮動基準SW、U9ではGND。各電圧・基準は端子と接続を参照する。
      | 用語5　　　　　　　 ; SW：Switching Node（スイッチング点）。主電力段の上下MOSFETとL1がつながる、電圧が高速に切り替わる点。GNDとは別電位。
  Pin_019 : PMIOPort  Description=|  Port=36  Side=Right  ConnectionType=Connection: foundation.electrical.electrical
      | 識別名　　　　　　　; Pin_019
      | 種別　　　　　　　　; Simscape Connection Port（階層境界の物理端子）
      | 所属部品　　　　　　; U10
      | 配置目的　　　　　　; 内部の電気ノードを、この外箱の外側の対応端子へ引き出す。
      | 対応端子　　　　　　; rconn:1／19番 VEE
      | 接続ラベル　　　　　; ラベルなし。接続は実線と境界対応で定義する。
      | モデルの範囲　　　　; 実部品を1個追加する表現ではない。端子自体に増幅・遮断・測定機能を持たない。
      | 端子番号の注意　　　; Connection Portの番号は外箱内の対応番号であり、実パッケージのピン番号とは区別する。
      | 確認の範囲　　　　　; 実ポートと階層対応による静的接続の説明。電気特性の再現性は所属部品の説明を参照する。
      | 
      | 従来の補足　　　　　; 以前のDescriptionを以下に保持する。
      | Physical U10 pin 19 / VEE
      | 
      | 【この説明欄の略語・記号】
      | 用語1　　　　　　　 ; IC：Integrated Circuit（集積回路）。複数の電子素子と機能を小さな半導体チップに集積した部品。
      | 用語2　　　　　　　 ; MOSFET：Metal-Oxide-Semiconductor Field-Effect Transistor（金属・酸化膜・半導体構造の電界効果トランジスタ）。ゲートとソースの電圧でドレインとソースの導通を制御する素子。N-MOSはNチャネル型を表す。
      | 用語3　　　　　　　 ; GND：Ground（回路の基準電位・電流帰路）。この図の共通基準。保護接地や大地への接続を意味するとは限らない。
      | 用語4　　　　　　　 ; VCC/VDD/VEE/VS：ICの電源端子名。文字の歴史的な由来を現在の接続機能へ当てはめない。現回路のVEEはU8/U10では浮動基準SW、U9ではGND。各電圧・基準は端子と接続を参照する。
      | 用語5　　　　　　　 ; SW：Switching Node（スイッチング点）。主電力段の上下MOSFETとL1がつながる、電圧が高速に切り替わる点。GNDとは別電位。

== system solar_pv_protected_c07_circuit/U11 ==
  Pin_003 : PMIOPort  Description=|  Side=Left  ConnectionType=Connection: foundation.electrical.electrical
      | 識別名　　　　　　　; Pin_003
      | 種別　　　　　　　　; Simscape Connection Port（階層境界の物理端子）
      | 所属部品　　　　　　; U11
      | 配置目的　　　　　　; 内部の電気ノードを、この外箱の外側の対応端子へ引き出す。
      | 対応端子　　　　　　; lconn:3／4番 CASE
      | 接続ラベル　　　　　; ラベルなし。接続は実線と境界対応で定義する。
      | モデルの範囲　　　　; 実部品を1個追加する表現ではない。端子自体に増幅・遮断・測定機能を持たない。
      | 端子番号の注意　　　; Connection Portの番号は外箱内の対応番号であり、実パッケージのピン番号とは区別する。
      | 確認の範囲　　　　　; 実ポートと階層対応による静的接続の説明。電気特性の再現性は所属部品の説明を参照する。
      | 
      | 従来の補足　　　　　; 以前のDescriptionを以下に保持する。
      | Physical U11 pin 4 / CASE
  Pin_001 : PMIOPort  Description=|  Port=2  Side=Left  ConnectionType=Connection: foundation.electrical.electrical
      | 識別名　　　　　　　; Pin_001
      | 種別　　　　　　　　; Simscape Connection Port（階層境界の物理端子）
      | 所属部品　　　　　　; U11
      | 配置目的　　　　　　; 内部の電気ノードを、この外箱の外側の対応端子へ引き出す。
      | 対応端子　　　　　　; lconn:1／1番 +VIN
      | 接続ラベル　　　　　; BAT_AUX
      | モデルの範囲　　　　; 実部品を1個追加する表現ではない。端子自体に増幅・遮断・測定機能を持たない。
      | 端子番号の注意　　　; Connection Portの番号は外箱内の対応番号であり、実パッケージのピン番号とは区別する。
      | 確認の範囲　　　　　; 実ポートと階層対応による静的接続の説明。電気特性の再現性は所属部品の説明を参照する。
      | 
      | 従来の補足　　　　　; 以前のDescriptionを以下に保持する。
      | Physical U11 pin 1 / +VIN
      | 
      | 【この説明欄の略語・記号】
      | 用語1　　　　　　　 ; VIN/VOUT：入力電圧・出力電圧を表す端子／ネット名。INは入力、OUTは出力。電源変換器の電力端子なのか、検出用端子なのかは対象部品によって異なるため、端子と接続の説明に従う。
  Pin_002 : PMIOPort  Description=|  Port=3  Side=Left  ConnectionType=Connection: foundation.electrical.electrical
      | 識別名　　　　　　　; Pin_002
      | 種別　　　　　　　　; Simscape Connection Port（階層境界の物理端子）
      | 所属部品　　　　　　; U11
      | 配置目的　　　　　　; 内部の電気ノードを、この外箱の外側の対応端子へ引き出す。
      | 対応端子　　　　　　; lconn:2／2番 GND
      | 接続ラベル　　　　　; GND、PROT_RETURN
      | モデルの範囲　　　　; 実部品を1個追加する表現ではない。端子自体に増幅・遮断・測定機能を持たない。
      | 端子番号の注意　　　; Connection Portの番号は外箱内の対応番号であり、実パッケージのピン番号とは区別する。
      | 確認の範囲　　　　　; 実ポートと階層対応による静的接続の説明。電気特性の再現性は所属部品の説明を参照する。
      | 
      | 従来の補足　　　　　; 以前のDescriptionを以下に保持する。
      | Physical U11 pin 2 / GND
      | 
      | 【この説明欄の略語・記号】
      | 用語1　　　　　　　 ; GND：Ground（回路の基準電位・電流帰路）。この図の共通基準。保護接地や大地への接続を意味するとは限らない。
      | 用語2　　　　　　　 ; PROT_RETURN：保護回路の共通帰路。PROTはProtection（保護）、RETURNは帰路。プロトタイプの略ではなく、現回路では共通GNDへつながる。
  Pin_005 : PMIOPort  Description=|  Port=4  Side=Left  ConnectionType=Connection: foundation.electrical.electrical
      | 識別名　　　　　　　; Pin_005
      | 種別　　　　　　　　; Simscape Connection Port（階層境界の物理端子）
      | 所属部品　　　　　　; U11
      | 配置目的　　　　　　; 内部の電気ノードを、この外箱の外側の対応端子へ引き出す。
      | 対応端子　　　　　　; rconn:1／3番 +VOUT
      | 接続ラベル　　　　　; P12
      | モデルの範囲　　　　; 実部品を1個追加する表現ではない。端子自体に増幅・遮断・測定機能を持たない。
      | 端子番号の注意　　　; Connection Portの番号は外箱内の対応番号であり、実パッケージのピン番号とは区別する。
      | 確認の範囲　　　　　; 実ポートと階層対応による静的接続の説明。電気特性の再現性は所属部品の説明を参照する。
      | 
      | 従来の補足　　　　　; 以前のDescriptionを以下に保持する。
      | Physical U11 pin 3 / +VOUT
      | 
      | 【この説明欄の略語・記号】
      | 用語1　　　　　　　 ; VIN/VOUT：入力電圧・出力電圧を表す端子／ネット名。INは入力、OUTは出力。電源変換器の電力端子なのか、検出用端子なのかは対象部品によって異なるため、端子と接続の説明に従う。
  Pin_004 : PMIOPort  Description=|  Port=5  Side=Left  ConnectionType=Connection: foundation.electrical.electrical
      | 識別名　　　　　　　; Pin_004
      | 種別　　　　　　　　; Simscape Connection Port（階層境界の物理端子）
      | 所属部品　　　　　　; U11
      | 配置目的　　　　　　; 内部の電気ノードを、この外箱の外側の対応端子へ引き出す。
      | 対応端子　　　　　　; lconn:4／5番 CASE
      | 接続ラベル　　　　　; ラベルなし。接続は実線と境界対応で定義する。
      | モデルの範囲　　　　; 実部品を1個追加する表現ではない。端子自体に増幅・遮断・測定機能を持たない。
      | 端子番号の注意　　　; Connection Portの番号は外箱内の対応番号であり、実パッケージのピン番号とは区別する。
      | 確認の範囲　　　　　; 実ポートと階層対応による静的接続の説明。電気特性の再現性は所属部品の説明を参照する。
      | 
      | 従来の補足　　　　　; 以前のDescriptionを以下に保持する。
      | Physical U11 pin 5 / CASE

== system solar_pv_protected_c07_circuit/U12 ==
  Pin_001 : PMIOPort  Description=|  Side=Left  ConnectionType=Connection: foundation.electrical.electrical
      | 識別名　　　　　　　; Pin_001
      | 種別　　　　　　　　; Simscape Connection Port（階層境界の物理端子）
      | 所属部品　　　　　　; U12
      | 配置目的　　　　　　; 内部の電気ノードを、この外箱の外側の対応端子へ引き出す。
      | 対応端子　　　　　　; lconn:1／1番 +VIN
      | 接続ラベル　　　　　; P12
      | モデルの範囲　　　　; 実部品を1個追加する表現ではない。端子自体に増幅・遮断・測定機能を持たない。
      | 端子番号の注意　　　; Connection Portの番号は外箱内の対応番号であり、実パッケージのピン番号とは区別する。
      | 確認の範囲　　　　　; 実ポートと階層対応による静的接続の説明。電気特性の再現性は所属部品の説明を参照する。
      | 
      | 従来の補足　　　　　; 以前のDescriptionを以下に保持する。
      | Physical U12 pin 1 / +VIN
      | 
      | 【この説明欄の略語・記号】
      | 用語1　　　　　　　 ; VIN/VOUT：入力電圧・出力電圧を表す端子／ネット名。INは入力、OUTは出力。電源変換器の電力端子なのか、検出用端子なのかは対象部品によって異なるため、端子と接続の説明に従う。
  Pin_002 : PMIOPort  Description=|  Port=2  Side=Left  ConnectionType=Connection: foundation.electrical.electrical
      | 識別名　　　　　　　; Pin_002
      | 種別　　　　　　　　; Simscape Connection Port（階層境界の物理端子）
      | 所属部品　　　　　　; U12
      | 配置目的　　　　　　; 内部の電気ノードを、この外箱の外側の対応端子へ引き出す。
      | 対応端子　　　　　　; lconn:2／2番 GND
      | 接続ラベル　　　　　; GND、PROT_RETURN
      | モデルの範囲　　　　; 実部品を1個追加する表現ではない。端子自体に増幅・遮断・測定機能を持たない。
      | 端子番号の注意　　　; Connection Portの番号は外箱内の対応番号であり、実パッケージのピン番号とは区別する。
      | 確認の範囲　　　　　; 実ポートと階層対応による静的接続の説明。電気特性の再現性は所属部品の説明を参照する。
      | 
      | 従来の補足　　　　　; 以前のDescriptionを以下に保持する。
      | Physical U12 pin 2 / GND
      | 
      | 【この説明欄の略語・記号】
      | 用語1　　　　　　　 ; GND：Ground（回路の基準電位・電流帰路）。この図の共通基準。保護接地や大地への接続を意味するとは限らない。
      | 用語2　　　　　　　 ; PROT_RETURN：保護回路の共通帰路。PROTはProtection（保護）、RETURNは帰路。プロトタイプの略ではなく、現回路では共通GNDへつながる。
  Pin_003 : PMIOPort  Description=|  Port=3  Side=Left  ConnectionType=Connection: foundation.electrical.electrical
      | 識別名　　　　　　　; Pin_003
      | 種別　　　　　　　　; Simscape Connection Port（階層境界の物理端子）
      | 所属部品　　　　　　; U12
      | 配置目的　　　　　　; 内部の電気ノードを、この外箱の外側の対応端子へ引き出す。
      | 対応端子　　　　　　; rconn:1／3番 +VOUT
      | 接続ラベル　　　　　; P5
      | モデルの範囲　　　　; 実部品を1個追加する表現ではない。端子自体に増幅・遮断・測定機能を持たない。
      | 端子番号の注意　　　; Connection Portの番号は外箱内の対応番号であり、実パッケージのピン番号とは区別する。
      | 確認の範囲　　　　　; 実ポートと階層対応による静的接続の説明。電気特性の再現性は所属部品の説明を参照する。
      | 
      | 従来の補足　　　　　; 以前のDescriptionを以下に保持する。
      | Physical U12 pin 3 / +VOUT
      | 
      | 【この説明欄の略語・記号】
      | 用語1　　　　　　　 ; VIN/VOUT：入力電圧・出力電圧を表す端子／ネット名。INは入力、OUTは出力。電源変換器の電力端子なのか、検出用端子なのかは対象部品によって異なるため、端子と接続の説明に従う。
